simulink model "tb_impl_codec"  (R2026b)
model workspace (MAT data in the model file):
  TB.cmd = [0 0 0 0 0]
  TB.fb = [0 0 0 0 0 0 0 0 0]
undefined symbols (not defined in the file or in its folder): Ts
settings Model: Creator=aomar  LastModifiedBy=aomar

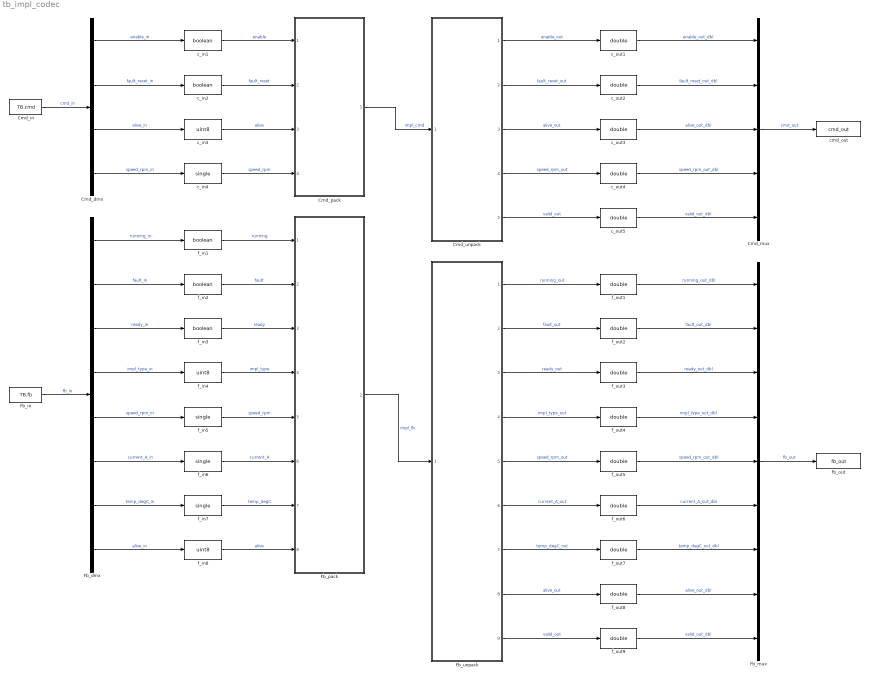
== system tb_impl_codec ==
  Cmd_dmx : Demux
  Cmd_in : FromWorkspace  VariableName=TB.cmd  SampleTime=Ts.can_slow  Interpolate=off  OutputAfterFinalValue=Holding final value
  Cmd_mux : Mux  Inputs=5
  Cmd_pack : Subsystem  ReferencedSubsystem=implcmd_can_pack
  Cmd_unpack : Subsystem  ReferencedSubsystem=implcmd_can_unpack
  Fb_dmx : Demux  Outputs=8
  Fb_in : FromWorkspace  VariableName=TB.fb  SampleTime=Ts.can_slow  Interpolate=off  OutputAfterFinalValue=Holding final value
  Fb_mux : Mux  Inputs=9
  Fb_pack : Subsystem  ReferencedSubsystem=implfb_can_pack
  Fb_unpack : Subsystem  ReferencedSubsystem=implfb_can_unpack
  c_in1 : DataTypeConversion  OutDataTypeStr=boolean  RndMeth=Nearest  SaturateOnIntegerOverflow=off
  c_in2 : DataTypeConversion  OutDataTypeStr=boolean  RndMeth=Nearest  SaturateOnIntegerOverflow=off
  c_in3 : DataTypeConversion  OutDataTypeStr=uint8  RndMeth=Nearest  SaturateOnIntegerOverflow=off
  c_in4 : DataTypeConversion  OutDataTypeStr=single  RndMeth=Nearest  SaturateOnIntegerOverflow=off
  c_out{1..5} (5 alike) : DataTypeConversion  OutDataTypeStr=double  SaturateOnIntegerOverflow=off  RndMeth=Floor
  cmd_out : ToWorkspace  VariableName=cmd_out  SampleTime=-1
  f_in1 : DataTypeConversion  OutDataTypeStr=boolean  RndMeth=Nearest  SaturateOnIntegerOverflow=off
  f_in2 : DataTypeConversion  OutDataTypeStr=boolean  RndMeth=Nearest  SaturateOnIntegerOverflow=off
  f_in3 : DataTypeConversion  OutDataTypeStr=boolean  RndMeth=Nearest  SaturateOnIntegerOverflow=off
  f_in4 : DataTypeConversion  OutDataTypeStr=uint8  RndMeth=Nearest  SaturateOnIntegerOverflow=off
  f_in5 : DataTypeConversion  OutDataTypeStr=single  RndMeth=Nearest  SaturateOnIntegerOverflow=off
  f_in6 : DataTypeConversion  OutDataTypeStr=single  RndMeth=Nearest  SaturateOnIntegerOverflow=off
  f_in7 : DataTypeConversion  OutDataTypeStr=single  RndMeth=Nearest  SaturateOnIntegerOverflow=off
  f_in8 : DataTypeConversion  OutDataTypeStr=uint8  RndMeth=Nearest  SaturateOnIntegerOverflow=off
  f_out{1..9} (9 alike) : DataTypeConversion  OutDataTypeStr=double  SaturateOnIntegerOverflow=off  RndMeth=Floor
  fb_out : ToWorkspace  VariableName=fb_out  SampleTime=-1
  wires:
  Cmd_in/1 -> Cmd_dmx/1  "cmd_in"
  Fb_in/1 -> Fb_dmx/1  "fb_in"
  Cmd_dmx/1 -> c_in1/1  "enable_in"
  Cmd_dmx/2 -> c_in2/1  "fault_reset_in"
  Cmd_dmx/3 -> c_in3/1  "alive_in"
  Cmd_dmx/4 -> c_in4/1  "speed_rpm_in"
  Fb_dmx/1 -> f_in1/1  "running_in"
  Fb_dmx/2 -> f_in2/1  "fault_in"
  Fb_dmx/3 -> f_in3/1  "ready_in"
  Fb_dmx/4 -> f_in4/1  "impl_type_in"
  Fb_dmx/5 -> f_in5/1  "speed_rpm_in"
  Fb_dmx/6 -> f_in6/1  "current_A_in"
  Fb_dmx/7 -> f_in7/1  "temp_degC_in"
  Fb_dmx/8 -> f_in8/1  "alive_in"
  c_in1/1 -> Cmd_pack/1  "enable"
  c_in2/1 -> Cmd_pack/2  "fault_reset"
  c_in3/1 -> Cmd_pack/3  "alive"
  c_in4/1 -> Cmd_pack/4  "speed_rpm"
  f_in1/1 -> Fb_pack/1  "running"
  f_in2/1 -> Fb_pack/2  "fault"
  f_in3/1 -> Fb_pack/3  "ready"
  f_in4/1 -> Fb_pack/4  "impl_type"
  f_in5/1 -> Fb_pack/5  "speed_rpm"
  f_in6/1 -> Fb_pack/6  "current_A"
  f_in7/1 -> Fb_pack/7  "temp_degC"
  f_in8/1 -> Fb_pack/8  "alive"
  Cmd_pack/1 -> Cmd_unpack/1  "impl_cmd"
  Fb_pack/1 -> Fb_unpack/1  "impl_fb"
  Cmd_unpack/1 -> c_out1/1  "enable_out"
  Cmd_unpack/2 -> c_out2/1  "fault_reset_out"
  Cmd_unpack/3 -> c_out3/1  "alive_out"
  Cmd_unpack/4 -> c_out4/1  "speed_rpm_out"
  Cmd_unpack/5 -> c_out5/1  "valid_out"
  Fb_unpack/1 -> f_out1/1  "running_out"
  Fb_unpack/2 -> f_out2/1  "fault_out"
  Fb_unpack/3 -> f_out3/1  "ready_out"
  Fb_unpack/4 -> f_out4/1  "impl_type_out"
  Fb_unpack/5 -> f_out5/1  "speed_rpm_out"
  Fb_unpack/6 -> f_out6/1  "current_A_out"
  Fb_unpack/7 -> f_out7/1  "temp_degC_out"
  Fb_unpack/8 -> f_out8/1  "alive_out"
  Fb_unpack/9 -> f_out9/1  "valid_out"
  c_out1/1 -> Cmd_mux/1  "enable_out_dbl"
  c_out2/1 -> Cmd_mux/2  "fault_reset_out_dbl"
  c_out3/1 -> Cmd_mux/3  "alive_out_dbl"
  c_out4/1 -> Cmd_mux/4  "speed_rpm_out_dbl"
  c_out5/1 -> Cmd_mux/5  "valid_out_dbl"
  f_out1/1 -> Fb_mux/1  "running_out_dbl"
  f_out2/1 -> Fb_mux/2  "fault_out_dbl"
  f_out3/1 -> Fb_mux/3  "ready_out_dbl"
  f_out4/1 -> Fb_mux/4  "impl_type_out_dbl"
  f_out5/1 -> Fb_mux/5  "speed_rpm_out_dbl"
  f_out6/1 -> Fb_mux/6  "current_A_out_dbl"
  f_out7/1 -> Fb_mux/7  "temp_degC_out_dbl"
  f_out8/1 -> Fb_mux/8  "alive_out_dbl"
  f_out9/1 -> Fb_mux/9  "valid_out_dbl"
  Cmd_mux/1 -> cmd_out/1  "cmd_out"
  Fb_mux/1 -> fb_out/1  "fb_out"
